simulink model "Leader_Follower"  (R2023a)
settings: Solver=VariableStepAuto  StartTime=0.0  StopTime=100  RelTol=1e-3
values from neighbouring files (symbols this model uses):
  follower1 = [-3, -3]    [DoiHinhDat.m]
  follower2 = [-3, 3]    [DoiHinhDat.m]
  P_pos_fl1 = 1    [Parameters.m]
  P_pos_fl2 = 1    [Parameters.m]
  P_pos_lead = 1    [Parameters.m]
  P_psi_fl1 = 2    [Parameters.m]
  P_psi_fl2 = 2    [Parameters.m]
  P_psi_lead = 2    [Parameters.m]
  P_vel_fl1 = 5    [Parameters.m]
  P_vel_fl2 = 5    [Parameters.m]
  P_vel_lead = 5    [Parameters.m]
  Waypoints_Matrix = [0, 50, 50, 0; 0, 0, 50, 50]    [Parameters.m]
libraries: uavalgslib x3
settings Model: Creator=NGOC MAI  LastModifiedBy=NGOC MAI

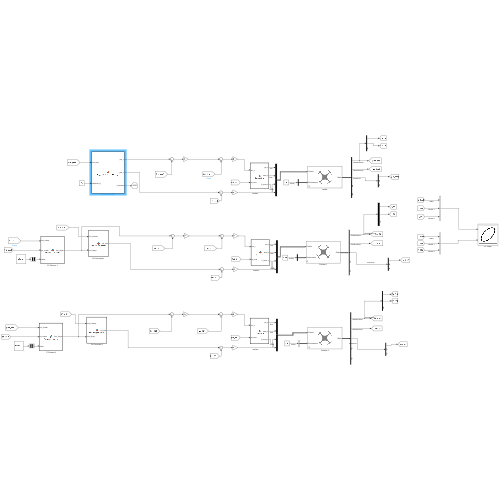
[thumbnail: Simulink's stored preview of the top-level diagram]
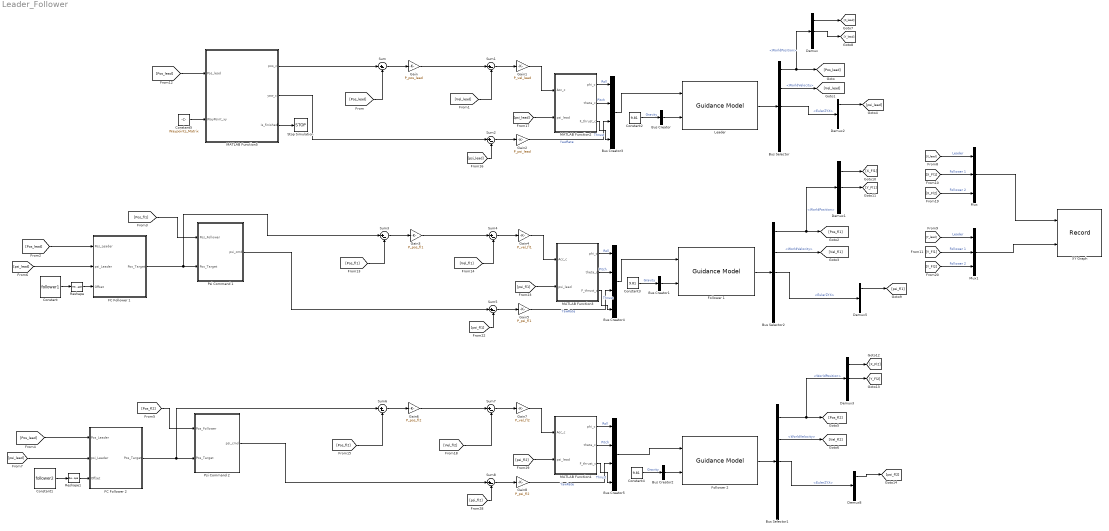
== system Leader_Follower ==
  Bus Creator : BusCreator  Inputs=1  OutDataTypeStr=Bus: MultirotorGuidanceEnvironmentBus  NonVirtualBus=on
  Bus Creator1 : BusCreator  Inputs=1  OutDataTypeStr=Bus: MultirotorGuidanceEnvironmentBus  NonVirtualBus=on
  Bus Creator2 : BusCreator  Inputs=1  OutDataTypeStr=Bus: MultirotorGuidanceEnvironmentBus  NonVirtualBus=on
  Bus Creator3 : BusCreator  Inputs=4  OutDataTypeStr=Bus: MultirotorGuidanceControlBus  NonVirtualBus=on
  Bus Creator4 : BusCreator  Inputs=4  OutDataTypeStr=Bus: MultirotorGuidanceControlBus  NonVirtualBus=on
  Bus Creator5 : BusCreator  Inputs=4  OutDataTypeStr=Bus: MultirotorGuidanceControlBus  NonVirtualBus=on
  Bus Selector : BusSelector  OutputSignals=WorldPosition,WorldVelocity,EulerZYX,BodyAngularRateRPY,Thrust
  Bus Selector1 : BusSelector  OutputSignals=WorldPosition,WorldVelocity,EulerZYX,BodyAngularRateRPY,Thrust
  Bus Selector2 : BusSelector  OutputSignals=WorldPosition,WorldVelocity,EulerZYX,BodyAngularRateRPY,Thrust
  Constant : Constant  Value=follower1
  Constant1 : Constant  Value=follower2
  Constant2 : Constant  Value=9.81
  Constant3 : Constant  Value=9.81
  Constant4 : Constant  Value=9.81
  Constant5 : Constant  Value=Waypoints_Matrix
  Demux{,1..3,5,8} (6 alike) : Demux  Outputs=3
  FC Follower 1 : MATLAB Function  TreatAsAtomicUnit=on
  FC Follower 2 : MATLAB Function  TreatAsAtomicUnit=on
  Follower 1 : uavalgslib/Guidance Model  ModelType=MultirotorGuidance  SpecifiedDataType=double  SimulateUsing=Interpreted execution  InitialWorldPositionMultirotor=[-5; 3; 5]  InitialWorldVelocityMultirotor=[0; 0; 0]  InitialEulerZYXMultirotor=[0; 0; 0]  InitialBodyAngularRateRPYMultirotor=[0; 0; 0]  InitialThrustMultirotor=0  InitialNorthFixedWing=0  InitialEastFixedWing=0  InitialHeightFixedWing=0  InitialAirSpeedFixedWing=0  InitialHeadingAngleFixedWing=0  InitialFlightPathAngleFixedWing=0  InitialRollAngleFixedWing=0  InitialRollAngleRateFixedWing=0  PDRollMultirotor=[3402.97,116.67]  PDPitchMultirotor=[3402.97, 116.67]  PYawRateMultirotor=1950  PThrustMultirotor=3900  MassMultirotor=0.1  PHeightFixedWing=3.9  PHeadingAngleFixedWing=3.9  PFlightPathAngleFixedWing=39  PDRollFixedWing=[3402.97, 116.67]  PAirSpeedFixedWing=1  FlightPathAngleLimitsFixedWing=[-pi/2, pi/2]  StateBusName='MultirotorGuidanceStateBus'  ControlBusName='MultirotorGuidanceControlBus'  EnvironmentBusName='MultirotorGuidanceEnvironmentBus'  DataType=double
  Follower 2 : uavalgslib/Guidance Model  ModelType=MultirotorGuidance  SpecifiedDataType=double  SimulateUsing=Interpreted execution  InitialWorldPositionMultirotor=[2; -4; 5]  InitialWorldVelocityMultirotor=[0; 0; 0]  InitialEulerZYXMultirotor=[0; 0; 0]  InitialBodyAngularRateRPYMultirotor=[0; 0; 0]  InitialThrustMultirotor=0  InitialNorthFixedWing=0  InitialEastFixedWing=0  InitialHeightFixedWing=0  InitialAirSpeedFixedWing=0  InitialHeadingAngleFixedWing=0  InitialFlightPathAngleFixedWing=0  InitialRollAngleFixedWing=0  InitialRollAngleRateFixedWing=0  PDRollMultirotor=[3402.97,116.67]  PDPitchMultirotor=[3402.97, 116.67]  PYawRateMultirotor=1950  PThrustMultirotor=3900  MassMultirotor=0.1  PHeightFixedWing=3.9  PHeadingAngleFixedWing=3.9  PFlightPathAngleFixedWing=39  PDRollFixedWing=[3402.97, 116.67]  PAirSpeedFixedWing=1  FlightPathAngleLimitsFixedWing=[-pi/2, pi/2]  StateBusName='MultirotorGuidanceStateBus'  ControlBusName='MultirotorGuidanceControlBus'  EnvironmentBusName='MultirotorGuidanceEnvironmentBus'  DataType=double
  Gain : Gain  Gain=P_pos_lead
  Gain1 : Gain  Gain=P_vel_lead
  Gain2 : Gain  Gain=P_psi_lead
  Gain3 : Gain  Gain=P_pos_fl1
  Gain4 : Gain  Gain=P_vel_fl1
  Gain5 : Gain  Gain=P_psi_fl1
  Gain6 : Gain  Gain=P_pos_fl2
  Gain7 : Gain  Gain=P_vel_fl2
  Gain8 : Gain  Gain=P_psi_fl2
  Leader : uavalgslib/Guidance Model  ModelType=MultirotorGuidance  SpecifiedDataType=double  SimulateUsing=Interpreted execution  InitialWorldPositionMultirotor=[0; 0; 5]  InitialWorldVelocityMultirotor=[0; 0; 0]  InitialEulerZYXMultirotor=[0; 0; 0]  InitialBodyAngularRateRPYMultirotor=[0; 0; 0]  InitialThrustMultirotor=0  InitialNorthFixedWing=0  InitialEastFixedWing=0  InitialHeightFixedWing=0  InitialAirSpeedFixedWing=0  InitialHeadingAngleFixedWing=0  InitialFlightPathAngleFixedWing=0  InitialRollAngleFixedWing=0  InitialRollAngleRateFixedWing=0  PDRollMultirotor=[3402.97,116.67]  PDPitchMultirotor=[3402.97, 116.67]  PYawRateMultirotor=1950  PThrustMultirotor=3900  MassMultirotor=0.1  PHeightFixedWing=3.9  PHeadingAngleFixedWing=3.9  PFlightPathAngleFixedWing=39  PDRollFixedWing=[3402.97, 116.67]  PAirSpeedFixedWing=1  FlightPathAngleLimitsFixedWing=[-pi/2, pi/2]  StateBusName='MultirotorGuidanceStateBus'  ControlBusName='MultirotorGuidanceControlBus'  EnvironmentBusName='MultirotorGuidanceEnvironmentBus'  DataType=double
  MATLAB Function2 : MATLAB Function  TreatAsAtomicUnit=on
  MATLAB Function3 : MATLAB Function  TreatAsAtomicUnit=on
  MATLAB Function4 : MATLAB Function  TreatAsAtomicUnit=on
  MATLAB Function5 : MATLAB Function  TreatAsAtomicUnit=on
  Mux : Mux  Inputs=3
  Mux1 : Mux  Inputs=3
  Psi Command 1 : MATLAB Function  TreatAsAtomicUnit=on
  Psi Command 2 : MATLAB Function  TreatAsAtomicUnit=on
  Reshape : Reshape  OutputDimensionality=Column vector (2-D)
  Reshape1 : Reshape  OutputDimensionality=Column vector (2-D)
  Stop Simulation : Stop
  Sum{,1..8} (9 alike) : Sum  Inputs=|+-
  XY Graph : Record  FileSettingsInternal="{\"entries\":[{\"content\":{\"excelSettings\":{\"content\":{},\"type\":\"Streamout.ExcelSettings\"}},\"type\":\"Streamout.FileSettingStorage\",\"uuid\":\"4b1d58a7-dbb8-4c8d-847a-b44ab9125955\"}],\"packageUris\":[\"http://schema.mathworks.com/mf0/streamout_blocks/R2020a\"],\"version\":\"1.0\"}"  Layout=[1 1]  SignalsInternal="{\"entries\":[{\"content\":{\"signals\":[{\"content\":{\"blockPath\":[\"Leader_Follower/XY Graph\"],\"dimensions\":[3],\"domain\":\"Leader_Follower/XY Graph\",\"hasChildren\":true,\"lineColor\":\"#77ac30\",\"port\":1,\"sid\":[\"\"],\"signalID\":32203,\"signalName\":\"Mux\"},\"type\":\"RecordBlkView.Signal\",\"uuid\":\"c1b8a284-bb3a-4bdd-8974-a916e57bb75b\"},{\"content\":{\"blockPath\":[\"Leader_Follower/XY Graph\"],\"channel\":[1],\"dimensions\":[3],\"domain\":\"Leader_Follower/XY Graph\",\"lineColor\":\"#7e2f8e\",\"parentID\":32203,\"plots\":[1],\"port\":1,\"sid\":[\"\"],\"signalID\":32204,\"signalName\":\"Mux\"},\"type\":\"RecordBlkView.Signal\",\"uuid\":\"019e48dd-5f67-4df9-9a93-23370b556c3a\"},{\"content\":{\"blockPath\":[\"Leader_Follower/XY Graph\"],\"dimensions\":[3],\"domain\":\"Leader_Follower/XY Graph\",\"hasChildren\":true,\"lineColor\":\"#a2142f\",\"port\":2,\"sid\":[\"\"],\"signalID\":32208,\"signalName\":\"Mux1\"},\"type\":\"RecordBlkView.Signal\",\"uuid\":\"7b5fff6b-3841-41a6-a5f8-c459f7dadffb\"},{\"content\":{\"blockPath\":[\"Leader_Follower/XY Graph\"],\"channel\":[1],\"dimensions\":[3],\"domain\":\"Leader_Follower/XY Graph\",\"lineColor\":\"#7e2f8e\",\"parentID\":32208,\"plots\":[1],\"port\":2,\"sid\":[\"\"],\"signalID\":32209,\"signalName\":\"Mux1\"},\"type\":\"RecordBlkView.Signal\",\"uuid\":\"41063eb6-9442-4218-8d3c-db1f133fb9d3\"},{\"content\":{\"blockPath\":[\"Leader_Follower/XY Graph\"],\"channel\":[2],\"dimensions\":[3],\"domain\":\"Leader_Follower/XY Graph\",\"lineColor\":\"#a2142f\",\"parentID\":32203,\"plots\":[1],\"port\":1,\"sid\":[\"\"],\"signalID\":32213,\"signalName\":\"Mux\"},\"type\":\"RecordBlkView.Signal\",\"uuid\":\"711e3b72-b1be-4628-be43-0ace20e96351\"},{\"content\":{\"blockPath\":[\"Leader_Follower/XY Graph\"],\"channel\":[3],\"dimensions\":[3],\"domain\":\"Leader_Follower/XY Graph\",\"lineColor\":\"#139fff\",\"parentID\":32203,\"plots\":[1],\"port\":1,\"sid\":[\"\"],\"signalID\":32214,\"signalName\":\"Mux\"},\"type\":\"RecordBlkView.Signal\",\"uuid\":\"0e4fce00-cb59-4e73-b721-d041ad73fef2\"},{\"content\":{\"blockPath\":[\"Leader_Follower/XY Graph\"],\"channel\":[2],\"dimensions\":[3],\"domain\":\"Leader_Follower/XY Graph\",\"lineColor\":\"#a2142f\",\"parentID\":32208,\"plots\":[1],\"port\":2,\"sid\":[\"\"],\"signalID\":32215,\"signalName\":\"Mux1\"},\"type\":\"RecordBlkView.Signal\",\"uuid\":\"70c55320-8f92-408d-8ea4-39646d50da28\"},{\"content\":{\"blockPath\":[\"Leader_Follower/XY Graph\"],\"channel\":[3],\"dimensions\":[3],\"domain\":\"Leader_Follower/XY Graph\",\"lineColor\":\"#139fff\",\"parentID\":32208,\"plots\":[1],\"port\":2,\"sid\":[\"\"],\"signalID\":32216,\"signalName\":\"Mux1\"},\"type\":\"RecordBlkView.Signal\",\"uuid\":\"ce29782b-732b-4125-9316-9719aa0e9e83\"}]},\"type\":\"RecordBlkView.InputSignals\",\"uuid\":\"868983d3-8f54-4d7c-b1c2-7dd08ac3f836\"}],\"packageUris\":[\"http://schema.mathworks.com/mf0/streamout_blocks/R2020a\"],\"version\":\"1.0\"}"  VisualizationBindings="{\"xyplotplugin\":{\"info\":[{\"series\":[{\"bindingParametersList\":[{\"parameter\":\"X-Axis\",\"signalID\":32204,\"signalName\":\"Mux(1)\"},{\"parameter\":\"Y-Axis\",\"signalID\":32209,\"signalName\":\"Mux1(1)\"}],\"seriesID\":17704},{\"bindingParametersList\":[{\"parameter\":\"X-Axis\",\"signalID\":32213,\"signalName\":\"Mux(2)\"},{\"parameter\":\"Y-Axis\",\"signalID\":32215,\"signalName\":\"Mux1(2)\"}],\"seriesID\":2079},{\"bindingParametersList\":[{\"parameter\":\"X-Axis\",\"signalID\":32214,\"signalName\":\"Mux(3)\"},{\"parameter\":\"Y-Axis\",\"signalID\":32216,\"signalName\":\"Mux1(3)\"}],\"seriesID\":39467}],\"subplotID\":1}]}}"  CompatibilityTag=XY
  wires:
  Constant/1 -> Reshape/1
  Constant1/1 -> Reshape1/1
  Reshape/1 -> FC Follower 1/3(Offset)
  Reshape1/1 -> FC Follower 2/3(Offset)
  Bus Creator/1 -> Leader/2
  Constant2/1 -> Bus Creator/1  "Gravity"
  Bus Creator1/1 -> Follower 1/2
  Constant3/1 -> Bus Creator1/1  "Gravity"
  Bus Creator2/1 -> Follower 2/2
  Constant4/1 -> Bus Creator2/1  "Gravity"
  FC Follower 1/1(Pos_Target) -> Sum3/1, Psi Command 1/2(Pos_Target)
  Follower 1/1 -> Bus Selector2/1
  Leader/1 -> Bus Selector/1
  Follower 2/1 -> Bus Selector1/1
  Bus Selector/3 -> Demux2/1  "<EulerZYX>"
  Demux2/1 -> [psi_lead]
  Demux5/1 -> [psi_fl1]
  Bus Selector2/3 -> Demux5/1  "<EulerZYX>"
  Demux8/1 -> [psi_fl2]
  Bus Selector1/3 -> Demux8/1  "<EulerZYX>"
  [psi_lead] -> FC Follower 1/2(psi_Leader)
  [psi_lead] -> FC Follower 2/2(psi_Leader)
  Gain1/1 -> MATLAB Function2/1(Acc_c)
  Bus Creator3/1 -> Leader/1
  MATLAB Function2/1(phi_c) -> Bus Creator3/1  "Roll"
  MATLAB Function2/2(theta_c) -> Bus Creator3/2  "Pitch"
  Sum1/1 -> Gain1/1
  Sum/1 -> Gain/1
  Sum2/1 -> Gain2/1
  [psi_lead] -> MATLAB Function2/2(psi_lead)
  [psi_lead] -> Sum2/2
  Gain/1 -> Sum1/1
  Bus Creator4/1 -> Follower 1/1
  Sum3/1 -> Gain3/1
  Gain4/1 -> MATLAB Function3/1(Acc_c)
  [psi_fl1] -> MATLAB Function3/2(psi_lead)
  [psi_fl1] -> Sum5/2
  MATLAB Function3/2(theta_c) -> Bus Creator4/2  "Pitch"
  MATLAB Function3/1(phi_c) -> Bus Creator4/1  "Roll"
  Gain3/1 -> Sum4/1
  Sum4/1 -> Gain4/1
  Sum5/1 -> Gain5/1
  Sum6/1 -> Gain6/1
  FC Follower 2/1(Pos_Target) -> Sum6/1, Psi Command 2/2(Pos_Target)
  Gain7/1 -> MATLAB Function4/1(Acc_c)
  [psi_fl2] -> MATLAB Function4/2(psi_lead)
  [psi_fl2] -> Sum8/2
  Gain6/1 -> Sum7/1
  Sum7/1 -> Gain7/1
  Sum8/1 -> Gain8/1
  MATLAB Function4/1(phi_c) -> Bus Creator5/1  "Roll"
  MATLAB Function4/2(theta_c) -> Bus Creator5/2  "Pitch"
  Bus Creator5/1 -> Follower 2/1
  Gain5/1 -> Bus Creator4/3  "YawRate"
  MATLAB Function3/3(F_thrust_c) -> Bus Creator4/4  "Thrust"
  Gain8/1 -> Bus Creator5/3  "YawRate"
  MATLAB Function4/3(F_thrust_c) -> Bus Creator5/4  "Thrust"
  Gain2/1 -> Bus Creator3/3  "YawRate"
  MATLAB Function2/3(F_thrust_c) -> Bus Creator3/4  "Thrust"
  Constant5/1 -> MATLAB Function5/2(WayPoint_xy)
  Bus Selector/1 -> Demux/1, [Pos_lead]  "<WorldPosition>"
  Bus Selector/2 -> [Vel_lead]  "<WorldVelocity>"
  [Pos_lead] -> Sum/2
  [Vel_lead] -> Sum1/2
  [Pos_lead] -> MATLAB Function5/1(Pos_lead)
  MATLAB Function5/1(pos_c) -> Sum/1
  MATLAB Function5/2(yaw_c) -> Sum2/1
  Bus Selector2/2 -> [Vel_fl1]  "<WorldVelocity>"
  [Pos_fl1] -> Sum3/2
  [Vel_fl1] -> Sum4/2
  Bus Selector1/2 -> [Vel_fl2]  "<WorldVelocity>"
  [Pos_fl2] -> Sum6/2
  [Vel_fl2] -> Sum7/2
  [Pos_lead] -> FC Follower 2/1(Pos_Leader)
  [Pos_fl2] -> Psi Command 2/1(Pos_Follower)
  [Pos_lead] -> FC Follower 1/1(Pos_Leader)
  [Pos_fl1] -> Psi Command 1/1(Pos_Follower)
  Psi Command 1/1(psi_cmd) -> Sum5/1
  Psi Command 2/1(psi_cmd) -> Sum8/1
  Bus Selector2/1 -> Demux1/1, [Pos_fl1]  "<WorldPosition>"
  Bus Selector1/1 -> Demux3/1, [Pos_fl2]  "<WorldPosition>"
  MATLAB Function5/3(is_finished) -> Stop Simulation/1
  Demux/1 -> [X_lead]
  Demux/2 -> [Y_lead]
  Demux1/1 -> [X_Fl1]
  Demux1/2 -> [Y_Fl1]
  Demux3/1 -> [X_Fl2]
  Demux3/2 -> [Y_Fl2]
  Mux1/1 -> XY Graph/2
  Mux/1 -> XY Graph/1
  [X_lead] -> Mux/1  "Leader"
  [Y_lead] -> Mux1/1  "Leader"
  [X_Fl1] -> Mux/2  "Follower 1"
  [Y_Fl1] -> Mux1/2  "Follower 1"
  [Y_Fl2] -> Mux1/3  "Follower 2"
  [X_Fl2] -> Mux/3  "Follower 2"

== matlab function Leader_Follower/FC Follower 1 ==
  data: Pos_Leader input; Pos_Target output; psi_Leader input; Offset input
function Pos_Target = Formation_Control(Pos_Leader, psi_Leader, Offset)
    % Offset: Vị trí tương đối [dx; dy] trong hệ tọa độ Leader
    % Pos_Leader: [x; y] từ Guidance Model của Leader
    % psi_Leader: Góc Yaw từ Guidance Model của Leader
    
    R_mat = [cos(psi_Leader), -sin(psi_Leader); 
             sin(psi_Leader),  cos(psi_Leader)];
         
    Pos_Target2D = Pos_Leader(1:2) + R_mat * Offset;
    Pos_Target = [Pos_Target2D(1); Pos_Target2D(2); Pos_Leader(3)];

end-

== matlab function Leader_Follower/FC Follower 2 ==
  data: Pos_Leader input; Pos_Target output; psi_Leader input; Offset input
function Pos_Target = Formation_Control(Pos_Leader, psi_Leader, Offset)
    % Offset: Vị trí tương đối [dx; dy] trong hệ tọa độ Leader
    % P_Leader: [x; y] từ Guidance Model của Leader
    % psi_Leader: Góc Yaw từ Guidance Model của Leader
    
    R_mat = [cos(psi_Leader), -sin(psi_Leader); 
             sin(psi_Leader),  cos(psi_Leader)];
         
        
    Pos_Target2D = Pos_Leader(1:2) + R_mat * Offset;
    Pos_Target = [Pos_Target2D(1); Pos_Target2D(2); Pos_Leader(3)];
end

== matlab function Leader_Follower/Psi Command 1 ==
  data: Pos_Follower input; psi_cmd output; Pos_Target input
function psi_cmd = Follower_Guidance(Pos_Follower, Pos_Target)
    % Pos_F: Vị trí hiện tại của Follower [x; y]
    % Pos_Target: Vị trí mục tiêu vừa tính từ khối Formation_Control [x; y]
    
    % Tính vector sai lệch vị trí (Delta)
    delta_x = Pos_Target(1) - Pos_Follower(1);
    delta_y = Pos_Target(2) - Pos_Follower(2);
    
    % Tính góc lệnh bằng atan2 (đảm bảo độ chính xác 4 góc phần tư)
    psi_cmd = atan2(delta_y, delta_x);
end

== matlab function Leader_Follower/Psi Command 2 ==
  data: Pos_Follower input; psi_cmd output; Pos_Target input
function psi_cmd = Follower_Guidance(Pos_Follower, Pos_Target)
    % Pos_F: Vị trí hiện tại của Follower [x; y]
    % Pos_Target: Vị trí mục tiêu vừa tính từ khối Formation_Control [x; y]
    
    % Tính vector sai lệch vị trí (Delta)
    delta_x = Pos_Target(1) - Pos_Follower(1);
    delta_y = Pos_Target(2) - Pos_Follower(2);
    
    % Tính góc lệnh bằng atan2 (đảm bảo độ chính xác 4 góc phần tư)
    psi_cmd = atan2(delta_y, delta_x);
end

== matlab function Leader_Follower/MATLAB Function2 ==
  data: Acc_c input; phi_c output; psi_lead input; theta_c output; F_thrust_c output
function [phi_c, theta_c, F_thrust_c] = Conversion(Acc_c, psi_lead)
    % Acc_c: Vector gia tốc mong muốn [ax; ay; az] từ bộ điều khiển P
    % psi: Góc Yaw hiện tại (rad)
    % m: Khối lượng UAV (kg)
    
    % Hằng số trọng trường
    g = 9.81;
    
    % Trích xuất các thành phần gia tốc
    ax = Acc_c(1);
    ay = Acc_c(2);
    az = Acc_c(3);
    
    % 1. Tính góc Roll lệnh (phi_c)
    % Công thức: 1/g * (ay * cos(psi) - ax * cos(psi))
    phi_c = (1/g) * (ay * cos(psi_lead) - ax * sin(psi_lead));
    
    % 2. Tính góc Pitch lệnh (theta_c)
    % Công thức: -1/g * (ax * cos(psi) + ay * sin(psi))
    theta_c = -(1/g) * (ax * cos(psi_lead) + ay * sin(psi_lead));
    
    % 3. Tính lực đẩy lệnh (F_thrust_c)
    % Công thức trong hệ NED: m * (g - az)
    % Lưu ý: Trong hệ NED, gia tốc az âm là hướng lên, dương là hướng xuống.
    F_thrust_c = 0.1 * (g - az);
    
    % Giới hạn giá trị (Safety Clamp) để tránh máy bay bị crash khi lệnh quá lớn
    phi_c = max(min(phi_c, deg2rad(45)), deg2rad(-45));
    theta_c = max(min(theta_c, deg2rad(45)), deg2rad(-45));
end

== matlab function Leader_Follower/MATLAB Function3 ==
  data: Acc_c input; phi_c output; psi_lead input; theta_c output; F_thrust_c output
function [phi_c, theta_c, F_thrust_c] = Conversion(Acc_c, psi_lead)
    % Acc_c: Vector gia tốc mong muốn [ax; ay; az] từ bộ điều khiển P
    % psi: Góc Yaw hiện tại (rad)
    % m: Khối lượng UAV (kg)
    
    % Hằng số trọng trường
    g = 9.81;
    
    % Trích xuất các thành phần gia tốc
    ax = Acc_c(1);
    ay = Acc_c(2);
    az = Acc_c(3);
    % 1. Tính góc Roll lệnh (phi_c)
    % Công thức: 1/g * (ay * cos(psi) - ax * cos(psi))
    phi_c = (1/g) * (ay * cos(psi_lead) - ax * sin(psi_lead));
    
    % 2. Tính góc Pitch lệnh (theta_c)
    % Công thức: -1/g * (ax * cos(psi) + ay * sin(psi))
    theta_c = -(1/g) * (ax * cos(psi_lead) + ay * sin(psi_lead));
    
    % 3. Tính lực đẩy lệnh (F_thrust_c)
    % Công thức trong hệ NED: m * (g - az)
    % Lưu ý: Trong hệ NED, gia tốc az âm là hướng lên, dương là hướng xuống.
    F_thrust_c = 0.1 * (g - az);
    
    % Giới hạn giá trị (Safety Clamp) để tránh máy bay bị crash khi lệnh quá lớn
    phi_c = max(min(phi_c, deg2rad(45)), deg2rad(-45));
    theta_c = max(min(theta_c, deg2rad(45)), deg2rad(-45));
end

== matlab function Leader_Follower/MATLAB Function4 ==
  data: Acc_c input; phi_c output; psi_lead input; theta_c output; F_thrust_c output
function [phi_c, theta_c, F_thrust_c] = Conversion(Acc_c, psi_lead)
    % Acc_c: Vector gia tốc mong muốn [ax; ay; az] từ bộ điều khiển P
    % psi: Góc Yaw hiện tại (rad)
    % m: Khối lượng UAV (kg)
    
    % Hằng số trọng trường
    g = 9.81;
    
    % Trích xuất các thành phần gia tốc
    ax = Acc_c(1);
    ay = Acc_c(2);
    az = Acc_c(3);
    % 1. Tính góc Roll lệnh (phi_c)
    % Công thức: 1/g * (ay * cos(psi) - ax * cos(psi))
    phi_c = (1/g) * (ay * cos(psi_lead) - ax * sin(psi_lead));
    
    % 2. Tính góc Pitch lệnh (theta_c)
    % Công thức: -1/g * (ax * cos(psi) + ay * sin(psi))
    theta_c = -(1/g) * (ax * cos(psi_lead) + ay * sin(psi_lead));
    
    % 3. Tính lực đẩy lệnh (F_thrust_c)
    % Công thức trong hệ NED: m * (g - az)
    % Lưu ý: Trong hệ NED, gia tốc az âm là hướng lên, dương là hướng xuống.
    F_thrust_c = 0.1 * (g - az);
    
    % Giới hạn giá trị (Safety Clamp) để tránh máy bay bị crash khi lệnh quá lớn
    phi_c = max(min(phi_c, deg2rad(45)), deg2rad(-45));
    theta_c = max(min(theta_c, deg2rad(45)), deg2rad(-45));
end

== matlab function Leader_Follower/MATLAB Function5 ==
  data: Pos_lead input; pos_c output; WayPoint_xy input; yaw_c output; is_finished output
function [pos_c, yaw_c, is_finished] = Waypoint_Follower_Manager(Pos_lead, WayPoint_xy)
    % Các tham số thiết kế
    R = 4.0;             % Khoảng cách nhìn trước (Look-ahead)
    Arrival_Radius = 2.0;     % Bán kính tiếp cận
    
    % Trích xuất tọa độ phẳng 2D
    Pos_lead2D = [Pos_lead(1); Pos_lead(2)];
    number_waypoint = size(WayPoint_xy, 2);
    
    % --- TÌM ĐOẠN ĐƯỜNG GẦN NHẤT ---
    min_dist = Inf;
    best_idx = 1;
    for i = 1:(number_waypoint - 1)
        W_A = WayPoint_xy(1:2, i);     
        W_B = WayPoint_xy(1:2, i+1);   
        V_line = W_B - W_A;
        u_line = V_line / norm(V_line);
        
        V_pos = Pos_lead2D - W_A;
        pro_len = dot(V_pos, u_line);
        pro_len = max(0, min(norm(V_line), pro_len));
        
        P_closest = W_A + pro_len * u_line;
        d = norm(Pos_lead2D - P_closest);
        
        if d < min_dist
            min_dist = d;
            best_idx = i;
        end
    end
    
    % --- TÍNH TOÁN ĐIỂM TARGET (Dựa trên W_A, W_B đã tìm được) ---
    W_A = WayPoint_xy(1:2, best_idx);
    W_B = WayPoint_xy(1:2, best_idx+1);
    
    V_line = W_B - W_A;
    u_line = V_line / norm(V_line);
    
    V_pos = Pos_lead2D - W_A;
    pro_len = dot(V_pos, u_line);
    P_H = W_A + pro_len * u_line;
    
    delta = sqrt(max(0, R^2 - min_dist^2));
    
    % Logic bo cua
    if (pro_len + delta > norm(W_B - W_A)) && (best_idx < number_waypoint - 1)
        W_next_start = WayPoint_xy(1:2, best_idx+1);
        W_next_end   = WayPoint_xy(1:2, best_idx+2);
        u_next = (W_next_end - W_next_start) / norm(W_next_end - W_next_start);
        remain_delta = (pro_len + delta) - norm(W_B - W_A);
        P_target = W_next_start + min(remain_delta, norm(W_next_end - W_next_start)) * u_next;
    else
        P_target = P_H + delta * u_line;
    end
    
    % --- KẾT QUẢ ĐẦU RA ---
    pos_c = [P_target(1); P_target(2); Pos_lead(3)]; % Giữ Z theo pos_curr
    err_vec = P_target - Pos_lead2D;
    yaw_c = atan2(err_vec(2), err_vec(1));
    
    % Kiểm tra hoàn thành
    dist_to_end = norm(Pos_lead2D - WayPoint_xy(1:2, end));
    is_finished = (dist_to_end < Arrival_Radius);
end
